simulink model "HorizontalControllerTest"  (R2026b)
settings: Solver=FixedStepDiscrete  StopTime=5  FixedStep=.0025
undefined symbols (not defined in the file): Heading, Height, HorizontalTestContext, HorizontalTestMotion, Position, Status, Velocity
settings Model: Creator=tyasukaw  LastModifiedBy=tyasukaw

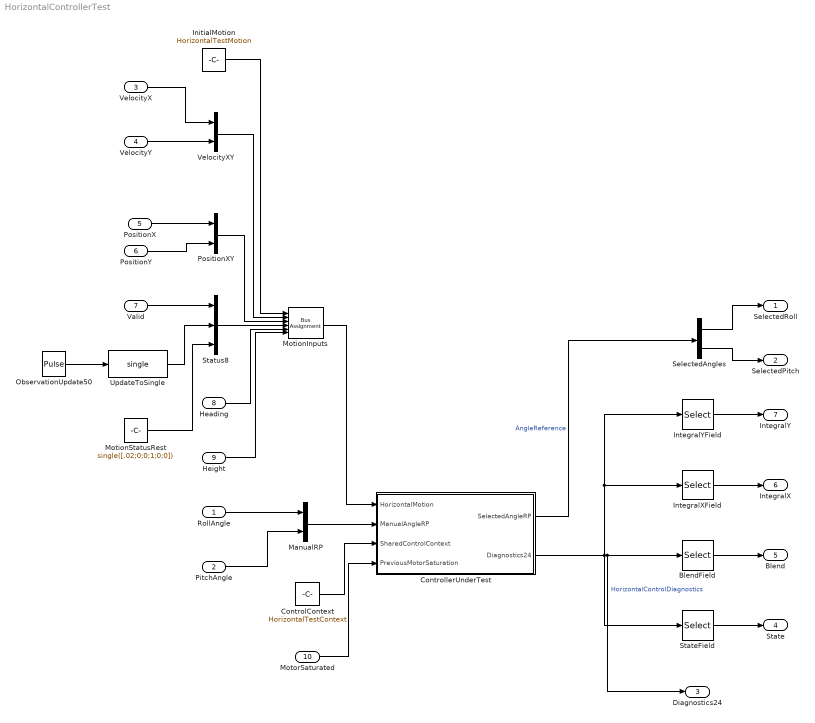
== system HorizontalControllerTest ==
  RollAngle : Inport  OutDataTypeStr=single  SampleTime=.0025
  PitchAngle : Inport  Port=2  OutDataTypeStr=single  SampleTime=.0025
  VelocityX : Inport  Port=3  OutDataTypeStr=single  SampleTime=.0025
  VelocityY : Inport  Port=4  OutDataTypeStr=single  SampleTime=.0025
  PositionX : Inport  Port=5  OutDataTypeStr=single  SampleTime=.0025
  PositionY : Inport  Port=6  OutDataTypeStr=single  SampleTime=.0025
  Valid : Inport  Port=7  OutDataTypeStr=single  SampleTime=.0025
  Heading : Inport  Port=8  OutDataTypeStr=single  SampleTime=.0025
  Height : Inport  Port=9  OutDataTypeStr=single  SampleTime=.0025
  MotorSaturated : Inport  Port=10  OutDataTypeStr=boolean  SampleTime=.0025
  BlendField : Selector  InputPortWidth=24  IndexOptions=Index vector (dialog)  Indices=15  OutputSizes=1
  ControlContext : Constant  Value=HorizontalTestContext  OutDataTypeStr=Bus: HorizontalControlContextBus
  ControllerUnderTest : Subsystem  Description=水平制御：移動・減速・停止位置保持の速度目標、速度PI、姿勢目標への変換を行います。既存の姿勢・角速度PIDの前段です。
      mask help: 水平制御：移動・減速・停止位置保持の速度目標、速度PI、姿勢目標への変換を行います。既存の姿勢・角速度PIDの前段です。
      mask Display: disp('HorizontalControl');port_label('input',1,'HorizontalMotion');port_label('input',2,'ManualAngleRP');port_label('input',3,'SharedControlContext');port_label('input',4,'PreviousMotorSaturation');port_label('output',1,'SelectedAngleRP');port_label('output',2,'Diagnostics24');
  InitialMotion : Constant  Value=HorizontalTestMotion  OutDataTypeStr=Bus: HorizontalMotionBus
  IntegralXField : Selector  InputPortWidth=24  IndexOptions=Index vector (dialog)  Indices=11  OutputSizes=1
  IntegralYField : Selector  InputPortWidth=24  IndexOptions=Index vector (dialog)  Indices=12  OutputSizes=1
  ManualRP : Mux  Inputs=2
  MotionInputs : BusAssignment  AssignedSignals=Velocity,Position,Status,Heading,Height
  MotionStatusRest : Constant  Value=single([.02;0;0;1;0;0])
  ObservationUpdate50 : DiscretePulseGenerator  PulseType=Time based  Period=.02  PulseWidth=12.5  PhaseDelay=.0175  SampleTime=.0025
  PositionXY : Mux  Inputs=2
  SelectedAngles : Demux  Outputs=2
  StateField : Selector  InputPortWidth=24  IndexOptions=Index vector (dialog)  Indices=16  OutputSizes=1
  Status8 : Mux  Inputs=3
  UpdateToSingle : DataTypeConversion  OutDataTypeStr=single  SaturateOnIntegerOverflow=off  RndMeth=Floor
  VelocityXY : Mux  Inputs=2
  SelectedRoll : Outport
  SelectedPitch : Outport  Port=2
  Diagnostics24 : Outport  Port=3
  State : Outport  Port=4
  Blend : Outport  Port=5
  IntegralX : Outport  Port=6
  IntegralY : Outport  Port=7
  wires:
  IntegralYField/1 -> IntegralY/1
  IntegralXField/1 -> IntegralX/1
  BlendField/1 -> Blend/1
  StateField/1 -> State/1
  ObservationUpdate50/1 -> UpdateToSingle/1
  UpdateToSingle/1 -> Status8/2
  RollAngle/1 -> ManualRP/1
  PitchAngle/1 -> ManualRP/2
  VelocityX/1 -> VelocityXY/1
  VelocityY/1 -> VelocityXY/2
  PositionX/1 -> PositionXY/1
  PositionY/1 -> PositionXY/2
  Valid/1 -> Status8/1
  MotionStatusRest/1 -> Status8/3
  InitialMotion/1 -> MotionInputs/1
  VelocityXY/1 -> MotionInputs/2
  PositionXY/1 -> MotionInputs/3
  Status8/1 -> MotionInputs/4
  Heading/1 -> MotionInputs/5
  Height/1 -> MotionInputs/6
  MotionInputs/1 -> ControllerUnderTest/1(HorizontalMotion)
  ManualRP/1 -> ControllerUnderTest/2(ManualAngleRP)
  ControlContext/1 -> ControllerUnderTest/3(SharedControlContext)
  MotorSaturated/1 -> ControllerUnderTest/4(PreviousMotorSaturation)
  ControllerUnderTest/1(SelectedAngleRP) -> SelectedAngles/1  "AngleReference"
  SelectedAngles/1 -> SelectedRoll/1
  SelectedAngles/2 -> SelectedPitch/1
  ControllerUnderTest/2(Diagnostics24) -> Diagnostics24/1, BlendField/1, IntegralXField/1, IntegralYField/1, StateField/1  "HorizontalControlDiagnostics"

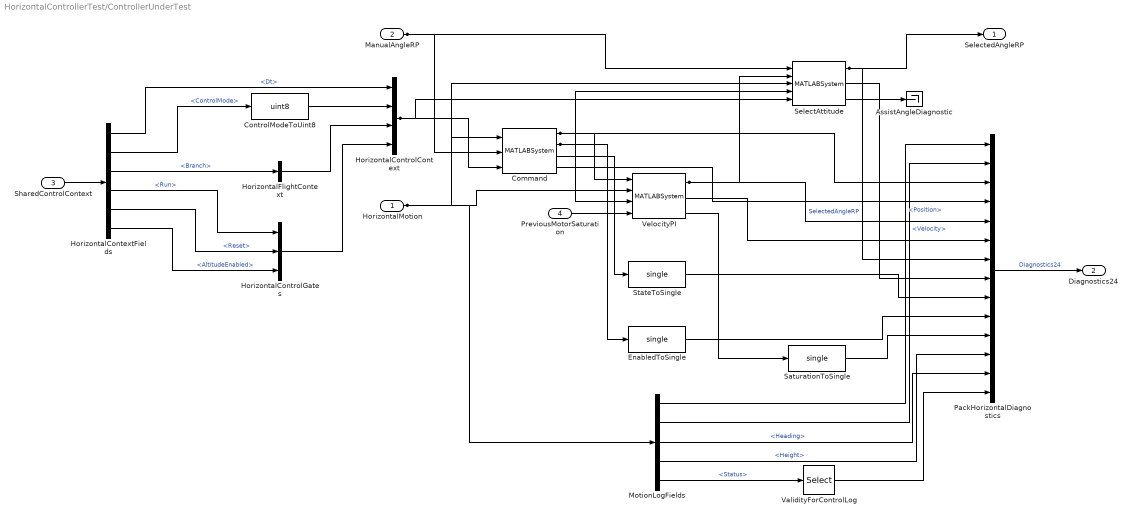
== system HorizontalControllerTest/ControllerUnderTest ==
  HorizontalMotion : Inport
  ManualAngleRP : Inport  Port=2
  SharedControlContext : Inport  Port=3
  PreviousMotorSaturation : Inport  Port=4
  AssistAngleDiagnostic : Terminator
  Command : MATLABSystem  System=horizontal.Command  Enabled=true  SampleTime=.0025  MaxSpeedMps=.3  CommandAccelerationMps2=.6  PositionGainPerS=.8  EngageHeightM=.20  ReleaseHeightM=.15  HealthyTimeS=.5  RecoveryTimeS=1.0  NeutralEnter=.05  NeutralExit=.08  StopSpeedMps=.08  StopTimeS=.3  ManualAngleLimitRad=pi / 6  SimulateUsing=Code generation
      mask Type: horizontal.Command
  ControlModeToUint8 : DataTypeConversion  OutDataTypeStr=uint8  SaturateOnIntegerOverflow=off  RndMeth=Floor
  EnabledToSingle : DataTypeConversion  OutDataTypeStr=single  SaturateOnIntegerOverflow=off  RndMeth=Floor
  HorizontalContextFields : BusSelector  OutputSignals=Dt,ControlMode,FlightContext.Branch,ControlContext.Run,ControlContext.Reset,ControlContext.AltitudeEnabled
  HorizontalControlContext : BusCreator  Inputs=4  OutDataTypeStr=Bus: HorizontalControlContextBus  NonVirtualBus=on
      settings: InheritFromInputs=off
  HorizontalControlGates : BusCreator  Inputs=3  OutDataTypeStr=Bus: HorizontalControlGatesBus  NonVirtualBus=on
      settings: InheritFromInputs=off
  HorizontalFlightContext : BusCreator  Inputs=1  OutDataTypeStr=Bus: HorizontalFlightContextBus  NonVirtualBus=on
      settings: InheritFromInputs=off
  MotionLogFields : BusSelector  OutputSignals=Position,Velocity,Heading,Height,Status
  PackHorizontalDiagnostics : Mux  Inputs=14
  SaturationToSingle : DataTypeConversion  OutDataTypeStr=single  SaturateOnIntegerOverflow=off  RndMeth=Floor
  SelectAttitude : MATLABSystem  System=horizontal.SelectAttitude  SampleTime=.0025  EngageTimeS=.3  ReleaseTimeS=.15  MaxAssistTiltDeg=10  MaxAssistTiltRateDegps=20  SimulateUsing=Code generation
      mask Type: horizontal.SelectAttitude
  StateToSingle : DataTypeConversion  OutDataTypeStr=single  SaturateOnIntegerOverflow=off  RndMeth=Floor
  ValidityForControlLog : Selector  InputPortWidth=8  IndexOptions=Index vector (dialog)  Indices=[1 4 5 7]  OutputSizes=1
  VelocityPI : MATLABSystem  System=horizontal.VelocityPI  SampleTime=.0025  ProportionalGainPerS=1.8  IntegralGainPerS2=.5  MaxAccelerationMps2=.6  IntegralLimitMps2=.25  AccelerationSlewMps3=2.0  SimulateUsing=Code generation
      mask Type: horizontal.VelocityPI
  SelectedAngleRP : Outport
  Diagnostics24 : Outport  Port=2
  wires:
  PackHorizontalDiagnostics/1 -> Diagnostics24/1  "Diagnostics24"
  ValidityForControlLog/1 -> PackHorizontalDiagnostics/14
  MotionLogFields/3 -> PackHorizontalDiagnostics/13  "<Heading>"
  MotionLogFields/4 -> PackHorizontalDiagnostics/12  "<Height>"
  SaturationToSingle/1 -> PackHorizontalDiagnostics/11
  EnabledToSingle/1 -> PackHorizontalDiagnostics/10
  StateToSingle/1 -> PackHorizontalDiagnostics/9
  SelectAttitude/2 -> PackHorizontalDiagnostics/8
  VelocityPI/2 -> PackHorizontalDiagnostics/6
  Command/4 -> PackHorizontalDiagnostics/4
  MotionLogFields/2 -> PackHorizontalDiagnostics/2  "<Velocity>"
  MotionLogFields/1 -> PackHorizontalDiagnostics/1  "<Position>"
  SelectAttitude/3 -> AssistAngleDiagnostic/1
  MotionLogFields/5 -> ValidityForControlLog/1  "<Status>"
  VelocityPI/3 -> SaturationToSingle/1
  Command/3 -> StateToSingle/1
  SelectAttitude/1 -> SelectedAngleRP/1, PackHorizontalDiagnostics/7  "SelectedAngleRP"
  VelocityPI/1 -> SelectAttitude/2, PackHorizontalDiagnostics/5
  PreviousMotorSaturation/1 -> VelocityPI/4
  Command/2 -> VelocityPI/3, SelectAttitude/4, EnabledToSingle/1
  Command/1 -> PackHorizontalDiagnostics/3, VelocityPI/1
  SharedControlContext/1 -> HorizontalContextFields/1
  ManualAngleRP/1 -> Command/2, SelectAttitude/1
  HorizontalMotion/1 -> MotionLogFields/1, VelocityPI/2, SelectAttitude/3, Command/1
  HorizontalContextFields/1 -> HorizontalControlContext/1  "<Dt>"
  HorizontalContextFields/2 -> ControlModeToUint8/1  "<ControlMode>"
  ControlModeToUint8/1 -> HorizontalControlContext/2
  HorizontalContextFields/3 -> HorizontalFlightContext/1  "<Branch>"
  HorizontalFlightContext/1 -> HorizontalControlContext/3
  HorizontalContextFields/4 -> HorizontalControlGates/1  "<Run>"
  HorizontalContextFields/5 -> HorizontalControlGates/2  "<Reset>"
  HorizontalContextFields/6 -> HorizontalControlGates/3  "<AltitudeEnabled>"
  HorizontalControlGates/1 -> HorizontalControlContext/4
  HorizontalControlContext/1 -> Command/3, SelectAttitude/5
